simulink model "LPsimulation"  (Simulink 7.0)
settings: Solver=FixedStepDiscrete  StartTime=0.0  StopTime=inf  FixedStep=1/300  RelTol=1e-3
undefined symbols (not defined in the file or in its folder): get
libraries: dspsigops x10, dspsnks4 x2, dspsrcs4 x1
settings Model: Creator=Casparus  LastModifiedBy=Casparus
settings OptimizationCC: InlineParams=on  InlineInvariantSignals=on  EnforceIntegerDowncast=off  ZeroExternalMemoryAtStartup=off  ZeroInternalMemoryAtStartup=off  InitFltsAndDblsToZero=off  EfficientFloat2IntCast=on  OptimizeModelRefInitCode=on  LifeSpan=1
settings DebuggingCC: SignalInfNanChecking=error  ReadBeforeWriteMsg=EnableAllAsError  WriteAfterWriteMsg=EnableAllAsError  WriteAfterReadMsg=EnableAllAsError  AlgebraicLoopMsg=error  ArtificialAlgebraicLoopMsg=error  CheckExecutionContextPreStartOutputMsg=on  CheckExecutionContextRuntimeOutputMsg=on  BlockPriorityViolationMsg=error  SolverPrmCheckMsg=error  InheritedTsInSrcMsg=error  DiscreteInheritContinuousMsg=error  SigSpecEnsureSampleTimeMsg=error  CheckMatrixSingularityMsg=error  IntegerOverflowMsg=error  ParameterUnderflowMsg=error  ParameterPrecisionLossMsg=error  ParameterTunabilityLossMsg=error  UnderSpecifiedDataTypeMsg=error  UnnecessaryDatatypeConvMsg=warning  VectorMatrixConversionMsg=error  FcnCallInpInsideContextMsg=Enable All  SignalLabelMismatchMsg=error  UnconnectedInputMsg=error  UnconnectedOutputMsg=error  UnconnectedLineMsg=error  SFcnCompatibilityMsg=error  BusObjectLabelMismatch=error  RootOutportRequireBusObject=error  AssertControl=DisableAll  ModelReferenceIOMsg=error  ModelReferenceIOMismatchMessage=error  ModelReferenceCSMismatchMessage=warning  UnknownTsInhSupMsg=error  ModelReferenceDataLoggingMessage=error
settings HardwareCC: ProdBitPerInt=16  ProdIntDivRoundTo=Floor  ProdEndianess=LittleEndian  ProdWordSize=16  ProdHWDeviceType=16-bit Generic  TargetHWDeviceType=32-bit Generic
settings RTWCC: SystemTargetFile=dspic.tlc  TemplateMakefile=dspic_pic30_gcc.tmf  PostCodeGenCommand=dsPIC_Compile()  Description=Embedded Target for Microchip dsPIC (real-time)  ProcessScript=dspic_make_rtw_hook
settings CodeAppCC: ForceParamTrailComments=on  IgnoreCustomStorageClasses=off  MangleLength=4  ReqsInCode=on
settings STFCustomTargetCC: GenFloatMathFcnCalls=ANSI_C  ModelReferenceCompliant=off  IncludeMdlTerminateFcn=off  CombineOutputUpdateFcns=on  SuppressErrorStatus=on  ERTCustomFileBanners=on  SupportNonFinite=off  SupportContinuousTime=off  SupportNonInlinedSFcns=off  SystemTargetFile=dspic.tlc
settings ERTTargetCC: GenFloatMathFcnCalls=ANSI_C  ModelReferenceCompliant=off  CompOptLevelCompliant=off  IncludeMdlTerminateFcn=off  SuppressErrorStatus=on  SupportNonFinite=off  ModelStepFunctionPrototypeControlCompliant=off  ExtModeMexFile=noextcomm  InlinedParameterPlacement=NonHierarchical  ERTSrcFileBannerTemplate=dsPIC_code_template.cgt  ERTHdrFileBannerTemplate=dsPIC_code_template.cgt  ERTDataSrcFileTemplate=dsPIC_code_template.cgt  ERTDataHdrFileTemplate=dsPIC_code_template.cgt  ERTCustomFileTemplate=dsPIC_main.tlc
settings CustomProperty: DataType=string  Value=C:\PROGRA~1\MATLAB\R2007b\bin\win32\gmake

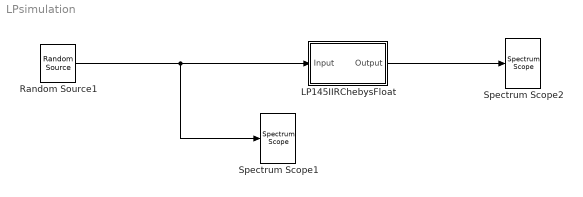
== system LPsimulation ==
  LP145IIRChebysFloat : Subsystem  Tag=FilterWizardSubSystem
      settings: ErrorFcn=dspFilterRealizedInBasicElemsAlgLoopErrFcnCallback
  Random Source1 : dspsrcs4/Random Source  SrcType=Gaussian  NormMethod=Ziggurat  CltLength=12  MinVal=0  MaxVal=1  MeanVal=0  VarVal=1  RepMode=Not repeatable  rawSeed=1  IsInherit=off  SampMode=Discrete  SampTime=1/300  SampFrame=1  DataType=Double  OutComplex=Real
  Spectrum Scope1 : dspsnks4/Spectrum Scope  DialogController=dspdialog.SpectrumScope  DialogControllerArgs=DataTag2  SystemSampleTime=-1  ScopeProperties=on  Domain=Frequency  HorizSpan=1  UseBuffer=on  BufferSize=128  Overlap=64  inpFftLenInherit=off  FFTlength=128  numAvg=2  DisplayProperties=off  AxisGrid=on  Memory=off  FrameNumber=on  AxisLegend=off  AxisZoom=off  OpenScopeAtSimStart=on  OpenScopeImmediately=off  FigPos=get(0,'defaultfigureposition')  AxisProperties=off  XUnits=Hertz  XRange=[0...Fs/2]  InheritXIncr=on  XIncr=1.0  XLabel=Samples  XLimit=Auto  YUnits=dB  XMax=1  XMin=0  YLabel=Magnitude-squared, dB  LineProperties=off  wintypeSpecScope=Hann  RsSpecScope=50  betaSpecScope=5  winsampSpecScope=Periodic
      settings: YMin=-23.2449567029934  YMax=8.31987938200619
  Spectrum Scope2 : dspsnks4/Spectrum Scope  DialogController=dspdialog.SpectrumScope  DialogControllerArgs=DataTag3  SystemSampleTime=-1  ScopeProperties=on  Domain=Frequency  HorizSpan=1  UseBuffer=on  BufferSize=128  Overlap=64  inpFftLenInherit=off  FFTlength=128  numAvg=2  DisplayProperties=off  AxisGrid=on  Memory=off  FrameNumber=on  AxisLegend=off  AxisZoom=off  OpenScopeAtSimStart=on  OpenScopeImmediately=off  FigPos=get(0,'defaultfigureposition')  AxisProperties=off  XUnits=Hertz  XRange=[0...Fs/2]  InheritXIncr=on  XIncr=1.0  XLabel=Samples  XLimit=Auto  YUnits=dB  XMax=1  XMin=0  YLabel=Magnitude-squared, dB  LineProperties=off  wintypeSpecScope=Hann  RsSpecScope=50  betaSpecScope=5  winsampSpecScope=Periodic
      settings: YMin=-58.8781484058797  YMax=9.65964313081179
  wires:
  LP145IIRChebysFloat/1(Output) -> Spectrum Scope2/1
  Random Source1/1 -> LP145IIRChebysFloat/1(Input), Spectrum Scope1/1

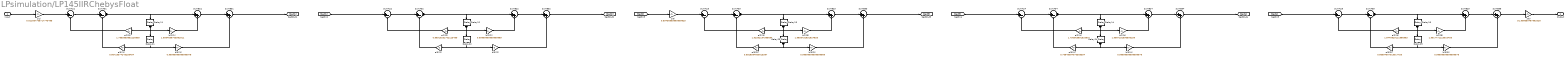
== system LPsimulation/LP145IIRChebysFloat ==
  Input : Inport
  Delay{11..15,21..25} (10 alike) : dspsigops/Delay  Orientation=down  dly_unit=Samples  delay=1  ic_detail=off  dif_ic_for_ch=off  dif_ic_for_dly=off  ic=0  reset_popup=None
  SumA{21..25,31..35} (10 alike) : Sum  Inputs=|+-  OutScaling=1  RndMeth=Nearest  SaturateOnIntegerOverflow=on
  SumB{21..25,31..35} (10 alike) : Sum  Inputs=|++  OutScaling=1  RndMeth=Nearest  SaturateOnIntegerOverflow=on
  a(2)(1) : Gain  Orientation=left  Gain=1.7855555852226805  ParameterDataTypeMode=Specify via dialog  ParameterDataType=float('double')  ParameterScalingMode=Use specified scaling  ParameterScaling=1  OutScaling=1  RndMeth=Nearest  SaturateOnIntegerOverflow=on
  a(2)(2) : Gain  Orientation=left  Gain=0.86910261702123459  ParameterDataTypeMode=Specify via dialog  ParameterDataType=float('double')  ParameterScalingMode=Use specified scaling  ParameterScaling=1  OutScaling=1  RndMeth=Nearest  SaturateOnIntegerOverflow=on
  a(2)(3) : Gain  Orientation=left  Gain=1.92352197385693  ParameterDataTypeMode=Specify via dialog  ParameterDataType=float('double')  ParameterScalingMode=Use specified scaling  ParameterScaling=1  OutScaling=1  RndMeth=Nearest  SaturateOnIntegerOverflow=on
  a(2)(4) : Gain  Orientation=left  Gain=1.750063891520601  ParameterDataTypeMode=Specify via dialog  ParameterDataType=float('double')  ParameterScalingMode=Use specified scaling  ParameterScaling=1  OutScaling=1  RndMeth=Nearest  SaturateOnIntegerOverflow=on
  a(2)(5) : Gain  Orientation=left  Gain=1.8440829111886963  ParameterDataTypeMode=Specify via dialog  ParameterDataType=float('double')  ParameterScalingMode=Use specified scaling  ParameterScaling=1  OutScaling=1  RndMeth=Nearest  SaturateOnIntegerOverflow=on
  a(3)(1) : Gain  Orientation=left  Gain=0.80725374243255454  ParameterDataTypeMode=Specify via dialog  ParameterDataType=float('double')  ParameterScalingMode=Use specified scaling  ParameterScaling=1  OutScaling=1  RndMeth=Nearest  SaturateOnIntegerOverflow=on
  a(3)(2) : Gain  Orientation=left  Gain=0  ParameterDataTypeMode=Specify via dialog  ParameterDataType=float('double')  ParameterScalingMode=Use specified scaling  ParameterScaling=1  OutScaling=1  RndMeth=Nearest  SaturateOnIntegerOverflow=on
  a(3)(3) : Gain  Orientation=left  Gain=0.9528594600013397  ParameterDataTypeMode=Specify via dialog  ParameterDataType=float('double')  ParameterScalingMode=Use specified scaling  ParameterScaling=1  OutScaling=1  RndMeth=Nearest  SaturateOnIntegerOverflow=on
  a(3)(4) : Gain  Orientation=left  Gain=0.76845094076305354  ParameterDataTypeMode=Specify via dialog  ParameterDataType=float('double')  ParameterScalingMode=Use specified scaling  ParameterScaling=1  OutScaling=1  RndMeth=Nearest  SaturateOnIntegerOverflow=on
  a(3)(5) : Gain  Orientation=left  Gain=0.86994907015017753  ParameterDataTypeMode=Specify via dialog  ParameterDataType=float('double')  ParameterScalingMode=Use specified scaling  ParameterScaling=1  OutScaling=1  RndMeth=Nearest  SaturateOnIntegerOverflow=on
  b(2)(1) : Gain  Gain=1.9954658703581811  ParameterDataTypeMode=Specify via dialog  ParameterDataType=float('double')  ParameterScalingMode=Use specified scaling  ParameterScaling=1  OutScaling=1  RndMeth=Nearest  SaturateOnIntegerOverflow=on
  b(2)(2) : Gain  Gain=0.99999999999999989  ParameterDataTypeMode=Specify via dialog  ParameterDataType=float('double')  ParameterScalingMode=Use specified scaling  ParameterScaling=1  OutScaling=1  RndMeth=Nearest  SaturateOnIntegerOverflow=on
  b(2)(3) : Gain  Gain=1.9893732831824833  ParameterDataTypeMode=Specify via dialog  ParameterDataType=float('double')  ParameterScalingMode=Use specified scaling  ParameterScaling=1  OutScaling=1  RndMeth=Nearest  SaturateOnIntegerOverflow=on
  b(2)(4) : Gain  Gain=1.9987152596506159  ParameterDataTypeMode=Specify via dialog  ParameterDataType=float('double')  ParameterScalingMode=Use specified scaling  ParameterScaling=1  OutScaling=1  RndMeth=Nearest  SaturateOnIntegerOverflow=on
  b(2)(5) : Gain  Gain=1.9917772123910493  ParameterDataTypeMode=Specify via dialog  ParameterDataType=float('double')  ParameterScalingMode=Use specified scaling  ParameterScaling=1  OutScaling=1  RndMeth=Nearest  SaturateOnIntegerOverflow=on
  b(3)(1) : Gain  Gain=0.99999999999999978  ParameterDataTypeMode=Specify via dialog  ParameterDataType=float('double')  ParameterScalingMode=Use specified scaling  ParameterScaling=1  OutScaling=1  RndMeth=Nearest  SaturateOnIntegerOverflow=on
  b(3)(2) : Gain  Gain=0  ParameterDataTypeMode=Specify via dialog  ParameterDataType=float('double')  ParameterScalingMode=Use specified scaling  ParameterScaling=1  OutScaling=1  RndMeth=Nearest  SaturateOnIntegerOverflow=on
  b(3)(3) : Gain  Gain=0.99999999999999989  ParameterDataTypeMode=Specify via dialog  ParameterDataType=float('double')  ParameterScalingMode=Use specified scaling  ParameterScaling=1  OutScaling=1  RndMeth=Nearest  SaturateOnIntegerOverflow=on
  b(3)(4) : Gain  Gain=0.99999999999999978  ParameterDataTypeMode=Specify via dialog  ParameterDataType=float('double')  ParameterScalingMode=Use specified scaling  ParameterScaling=1  OutScaling=1  RndMeth=Nearest  SaturateOnIntegerOverflow=on
  b(3)(5) : Gain  Gain=0.99999999999999978  ParameterDataTypeMode=Specify via dialog  ParameterDataType=float('double')  ParameterScalingMode=Use specified scaling  ParameterScaling=1  OutScaling=1  RndMeth=Nearest  SaturateOnIntegerOverflow=on
  s(1) : Gain  Gain=0.021667765717743495  ParameterDataTypeMode=Specify via dialog  ParameterDataType=float('double')  ParameterScalingMode=Use specified scaling  ParameterScaling=1  OutScaling=1  RndMeth=Nearest  SaturateOnIntegerOverflow=on
  s(3) : Gain  Gain=0.59436893860809825  ParameterDataTypeMode=Specify via dialog  ParameterDataType=float('double')  ParameterScalingMode=Use specified scaling  ParameterScaling=1  OutScaling=1  RndMeth=Nearest  SaturateOnIntegerOverflow=on
  s(6) : Gain  Gain=51.908650487962028  ParameterDataTypeMode=Specify via dialog  ParameterDataType=float('double')  ParameterScalingMode=Use specified scaling  ParameterScaling=1  OutScaling=1  RndMeth=Nearest  SaturateOnIntegerOverflow=on
  Output : Outport
  wires:
  s(6)/1 -> Output/1
  b(3)(5)/1 -> SumB35/2
  Delay25/1 -> b(3)(5)/1, a(3)(5)/1
  a(3)(5)/1 -> SumA35/2
  b(2)(5)/1 -> SumB25/2
  Delay15/1 -> Delay25/1, b(2)(5)/1, a(2)(5)/1
  a(2)(5)/1 -> SumA25/2
  SumB35/1 -> s(6)/1
  SumB25/1 -> SumB35/1
  SumA35/1 -> Delay15/1, SumB25/1
  SumA25/1 -> SumA35/1
  [Sect4] -> SumA25/1
  b(3)(4)/1 -> SumB34/2
  Delay24/1 -> b(3)(4)/1, a(3)(4)/1
  a(3)(4)/1 -> SumA34/2
  b(2)(4)/1 -> SumB24/2
  Delay14/1 -> Delay24/1, b(2)(4)/1, a(2)(4)/1
  a(2)(4)/1 -> SumA24/2
  SumB34/1 -> [Sect4]
  SumB24/1 -> SumB34/1
  SumA34/1 -> Delay14/1, SumB24/1
  SumA24/1 -> SumA34/1
  [Sect3] -> SumA24/1
  b(3)(3)/1 -> SumB33/2
  Delay23/1 -> b(3)(3)/1, a(3)(3)/1
  a(3)(3)/1 -> SumA33/2
  b(2)(3)/1 -> SumB23/2
  Delay13/1 -> Delay23/1, b(2)(3)/1, a(2)(3)/1
  a(2)(3)/1 -> SumA23/2
  SumB33/1 -> [Sect3]
  SumB23/1 -> SumB33/1
  SumA33/1 -> Delay13/1, SumB23/1
  SumA23/1 -> SumA33/1
  s(3)/1 -> SumA23/1
  [Sect2] -> s(3)/1
  b(3)(2)/1 -> SumB32/2
  Delay22/1 -> b(3)(2)/1, a(3)(2)/1
  a(3)(2)/1 -> SumA32/2
  b(2)(2)/1 -> SumB22/2
  Delay12/1 -> Delay22/1, b(2)(2)/1, a(2)(2)/1
  a(2)(2)/1 -> SumA22/2
  SumB32/1 -> [Sect2]
  SumB22/1 -> SumB32/1
  SumA32/1 -> Delay12/1, SumB22/1
  SumA22/1 -> SumA32/1
  [Sect1] -> SumA22/1
  b(3)(1)/1 -> SumB31/2
  Delay21/1 -> b(3)(1)/1, a(3)(1)/1
  a(3)(1)/1 -> SumA31/2
  b(2)(1)/1 -> SumB21/2
  Delay11/1 -> Delay21/1, b(2)(1)/1, a(2)(1)/1
  a(2)(1)/1 -> SumA21/2
  SumB31/1 -> [Sect1]
  SumB21/1 -> SumB31/1
  SumA31/1 -> Delay11/1, SumB21/1
  SumA21/1 -> SumA31/1
  s(1)/1 -> SumA21/1
  Input/1 -> s(1)/1
